simulink model "Accelero_Gyro_Combo_Lubins_Kalman"  (Simulink 7.0)
settings: Solver=FixedStepDiscrete  StartTime=0.0  StopTime=10.0  FixedStep=0.001  RelTol=1e-3
undefined symbols (not defined in the file or in its folder): Az, DiscIntNeverNeededParam, Kz, Ts
libraries: dsPICdrivers x6
settings Model: Creator=Lubin  LastModifiedBy=Prezes
settings OptimizationCC: OptimizeModelRefInitCode=on  LifeSpan=1
settings DebuggingCC: SaveWithParameterizedLinksMsg=none  SignalResolutionControl=TryResolveAllWithWarning
settings HardwareCC: ProdBitPerInt=16  ProdEndianess=LittleEndian  ProdWordSize=16  ProdHWDeviceType=16-bit Generic  TargetHWDeviceType=32-bit Generic
settings RTWCC: SystemTargetFile=dspic.tlc  TemplateMakefile=dspic_pic30_gcc.tmf  PostCodeGenCommand=dsPIC_Compile()  Description=Embedded Target for Microchip dsPIC (real-time)  ProcessScript=dspic_make_rtw_hook
settings CodeAppCC: IgnoreCustomStorageClasses=off
settings STFCustomTargetCC: GenFloatMathFcnCalls=ANSI_C  ModelReferenceCompliant=off  IncludeMdlTerminateFcn=off  CombineOutputUpdateFcns=on  SuppressErrorStatus=on  ERTCustomFileBanners=on  SupportContinuousTime=off  SupportNonInlinedSFcns=off  SystemTargetFile=dspic.tlc
settings ERTTargetCC: GenFloatMathFcnCalls=ANSI_C  ModelReferenceCompliant=off  CompOptLevelCompliant=off  IncludeMdlTerminateFcn=off  SuppressErrorStatus=on  ModelStepFunctionPrototypeControlCompliant=off  InlinedParameterPlacement=NonHierarchical  ERTSrcFileBannerTemplate=dsPIC_code_template.cgt  ERTHdrFileBannerTemplate=dsPIC_code_template.cgt  ERTDataSrcFileTemplate=dsPIC_code_template.cgt  ERTDataHdrFileTemplate=dsPIC_code_template.cgt  ERTCustomFileTemplate=dsPIC_main.tlc
settings CustomProperty: DataType=string  Value=D:\PROGRA~1\MATLAB\R2007b\bin\win32\gmake

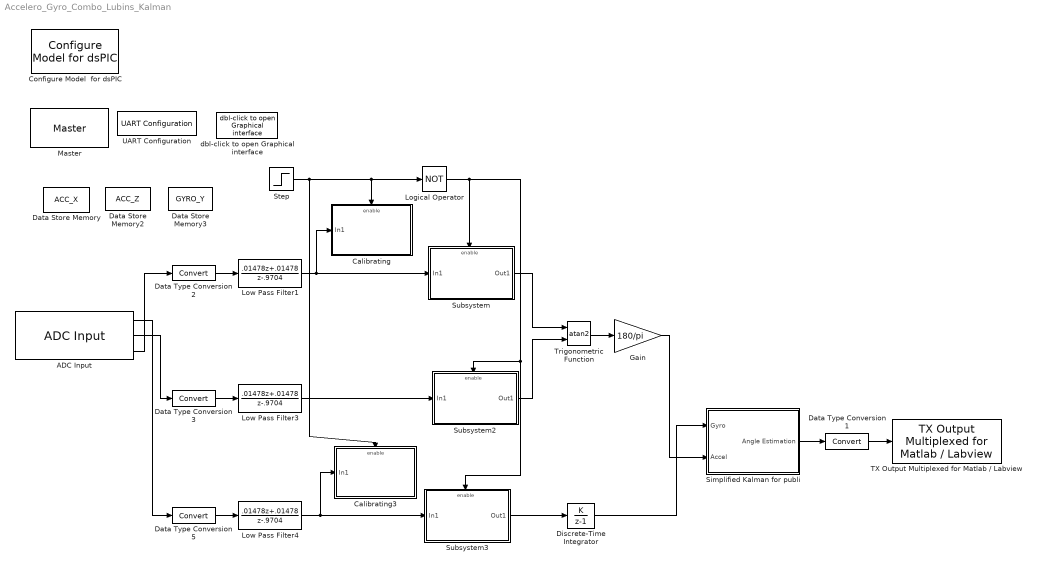
== system Accelero_Gyro_Combo_Lubins_Kalman ==
  ADC Input : dsPICdrivers/Peripheral I//O/ADC Input  Tag=dsPIC_ADC  Priority=5  ADC_TYPE=10 bits  ADC_MODE=Continuous sampling & get last channel value  NbrSampleStep=1  VoltRefpopup="AVdd  -  AVss"  OutFormatBitspopup=0000 00dd dddd dddd : Integer  InterruptPriority=6  ANCHANNELS=[11 14 15]  MaxName=ANmax = 1024  Rin=0  ADCS=3  SAMC=1  Temperature=25  DMAChannel=0  SampleTime=0.001  Status="OK  |  Tsmp=2.000e-007 |  T/Channel=2.600e-006 |  Tall=7.800e-006"
  Calibrating : Subsystem
  Calibrating3 : Subsystem
  Configure Model  for dsPIC : dsPICdrivers/Simulink Configuration/Configure Model  for dsPIC
  Data Store Memory : DataStoreMemory  DataStoreName=ACC_X  ReadBeforeWriteMsg=warning  WriteAfterWriteMsg=warning  WriteAfterReadMsg=warning  InitialValue=-1  OutDataType=sfix(16)  OutScaling=2^0
  Data Store Memory2 : DataStoreMemory  DataStoreName=ACC_Z  ReadBeforeWriteMsg=warning  WriteAfterWriteMsg=warning  WriteAfterReadMsg=warning  InitialValue=347  OutDataType=sfix(16)  OutScaling=2^0
  Data Store Memory3 : DataStoreMemory  DataStoreName=GYRO_Y  ReadBeforeWriteMsg=warning  WriteAfterWriteMsg=warning  WriteAfterReadMsg=warning  InitialValue=347  OutDataType=sfix(16)  OutScaling=2^0
  Data Type Conversion1 : DataTypeConversion  OutDataTypeMode=int16  OutDataType=sfix(16)  OutScaling=2^0
  Data Type Conversion2 : DataTypeConversion  OutDataTypeMode=double  OutDataType=sfix(16)  OutScaling=2^0
  Data Type Conversion3 : DataTypeConversion  OutDataTypeMode=double  OutDataType=sfix(16)  OutScaling=2^0
  Data Type Conversion5 : DataTypeConversion  OutDataTypeMode=double  OutDataType=sfix(16)  OutScaling=2^0
  Discrete-Time Integrator : DiscreteIntegrator  IntegratorMethod=Accumulation: Forward Euler  SampleTime=-1  OutDataTypeMode=double  OutDataType=sfix(16)  OutScaling=2^0  ICPrevOutput=DiscIntNeverNeededParam  ICPrevScaledInput=DiscIntNeverNeededParam
  Gain : Gain  Gain=180/pi  ParameterDataType=sfix(16)  ParameterScaling=2^0  OutDataTypeMode=double  OutDataType=sfix(16)  OutScaling=2^0
  Logical Operator : Logic  Operator=NOT  Inputs=1  AllPortsSameDT=off  OutDataTypeMode=boolean
  Low Pass Filter1 : DiscreteTransferFcn  Numerator=[.01478 .01478]  Denominator=[1 -.9704]  SampleTime=.001
  Low Pass Filter3 : DiscreteTransferFcn  Numerator=[.01478 .01478]  Denominator=[1 -.9704]  SampleTime=.001
  Low Pass Filter4 : DiscreteTransferFcn  Numerator=[.01478 .01478]  Denominator=[1 -.9704]  SampleTime=.001
  Master : dsPICdrivers/Master  Tag=dsPIC_MASTER  Priority=1  TimeStepType=Timer1  picType=30f6010A  fcy=10e6  Quartz_33f=5e6  PLLActive_33f=off  fcyDesired_33f=0  tmr1="[1  9999  0]"  tmr1Info="Time Step : 0.001  ;   Error : 0%  PR1=9999"  tmr2345="[0  0  0  0]"  tmr2345cfg=[-1 -1 -1 -1]  IOautoConf=on  typePort="[ 0  0  0  0  0  0  0  0  0  0  0  0  0  0  0  0  0  0  0  0  0  0  0  0  0  0  0  8  0  0  8  8  0  0  0  0  0  0  0  0  0  0  0  0  0  0  0  0  0  0  0  0  0  0  0  0  0  0  0  0  0  0  0  0  0  0  0  0  0  0  0  0  0  0  0  0  0  0  0  0  0  0  4  5  0  0  0  0  0  0  0  0  0  0  0  0  0  0  0  0  0  0  0  0  0  0  0  0  0  0  0  0 ]"  TRIS="[ 65535  65535  65535  65535  65535  65535  65535 ]"  ADPCFG=0  MasterBusyPort=None  MasterOverloadPort=None  FOSC=ECIO  TempProtection_33f=TEMP_ON  FPBOR=PBOR_OFF  PWRT=PWRT_OFF  MCLR=MCLR_DIS  PowerSave=off
  Simplified Kalman for publi : Subsystem
  Step : Step  Time=5  Before=1  After=0
  Subsystem : Subsystem
  Subsystem2 : Subsystem
  Subsystem3 : Subsystem
  TX Output Multiplexed for Matlab / Labview : dsPICdrivers/Serial PORT/TX Output Multiplexed for Matlab // Labview  Tag=dsPIC_TX_Multiplexed  Priority=5  UART=1  CleverSpreadingChk=on  CleverSpreading=1  CHANNEL=[0 ]  CHANNELBLOCKED=[]  CHANNELBLOCKED_BITEWISE=0  Status=OK
  Trigonometric Function : Trigonometry  Operator=atan2
  UART Configuration : dsPICdrivers/Serial PORT/UART Configuration  Tag=dsPIC_config_UART  Priority=2  UART=1  proposed_BAUD=9600  ALT_TX_RX=off  InterruptTxWhen=When Transmit Buffer is empty  TXInterruptPri=1  TxBufferSize=32  TXEN=on  InterruptRxWhen=When Receive Buffer is full (contain 4 characters)  RXInterruptPri=1  RxBufferSize=32  BAUD=9600  UxBRG=64  Info="UxBRG = 64   ||  Real Baud : 9615   ||  % error : 0.16026  ||  max 0.96154 Bytes / Step"  RealBaud=0
  dbl-click to open Graphical interface : dsPICdrivers/Serial PORT/dbl-click to open Graphical interface  SystemSampleTime=-1  Nothing=0
  wires:
  Trigonometric Function/1 -> Gain/1
  Discrete-Time Integrator/1 -> Simplified Kalman for publi/1(Gyro)
  Data Type Conversion2/1 -> Low Pass Filter1/1
  Low Pass Filter1/1 -> Calibrating/1(In1), Subsystem/1(In1)
  Step/1 -> Calibrating/Enable, Logical Operator/1, Calibrating3/Enable
  Logical Operator/1 -> Subsystem/Enable, Subsystem2/Enable, Subsystem3/Enable
  Data Type Conversion3/1 -> Low Pass Filter3/1
  Low Pass Filter3/1 -> Subsystem2/1(In1)
  Subsystem/1(Out1) -> Trigonometric Function/1
  Subsystem2/1(Out1) -> Trigonometric Function/2
  Data Type Conversion5/1 -> Low Pass Filter4/1
  Low Pass Filter4/1 -> Subsystem3/1(In1), Calibrating3/1(In1)
  Subsystem3/1(Out1) -> Discrete-Time Integrator/1
  ADC Input/3 -> Data Type Conversion2/1
  ADC Input/1 -> Data Type Conversion5/1
  ADC Input/2 -> Data Type Conversion3/1
  Gain/1 -> Simplified Kalman for publi/2(Accel)
  Simplified Kalman for publi/1(Angle Estimation) -> Data Type Conversion1/1
  Data Type Conversion1/1 -> TX Output Multiplexed for Matlab / Labview/1

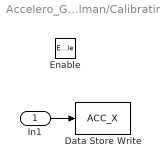
== system Accelero_Gyro_Combo_Lubins_Kalman/Calibrating ==
  In1 : Inport
  Enable : EnablePort  StatesWhenEnabling=reset
  Data Store Write : DataStoreWrite  DataStoreName=ACC_X  SampleTime=-1
  wires:
  In1/1 -> Data Store Write/1

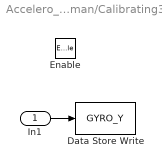
== system Accelero_Gyro_Combo_Lubins_Kalman/Calibrating3 ==
  In1 : Inport
  Enable : EnablePort  StatesWhenEnabling=reset
  Data Store Write : DataStoreWrite  DataStoreName=GYRO_Y  SampleTime=-1
  wires:
  In1/1 -> Data Store Write/1

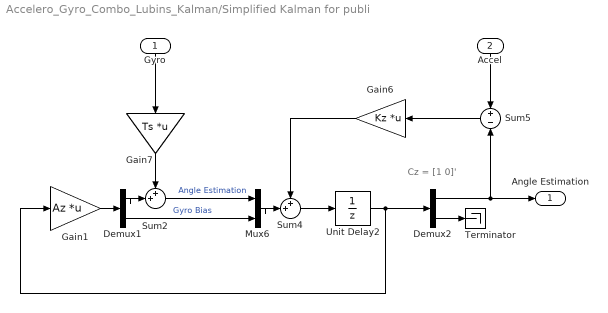
== system Accelero_Gyro_Combo_Lubins_Kalman/Simplified Kalman for publi ==
  note: Cz = [1 0]'
  Gyro : Inport  Orientation=down
  Accel : Inport  Orientation=down  Port=2
  Demux1 : Demux  Outputs=2
  Demux2 : Demux  Outputs=2
  Gain1 : Gain  Gain=Az  Multiplication=Matrix(K*u)  ParameterDataType=sfix(16)  ParameterScaling=2^0  OutDataType=sfix(16)  OutScaling=2^0
  Gain6 : Gain  Orientation=left  Gain=Kz  Multiplication=Matrix(K*u)  ParameterDataType=sfix(16)  ParameterScaling=2^0  OutDataType=sfix(16)  OutScaling=2^0
  Gain7 : Gain  Orientation=down  Gain=Ts  Multiplication=Matrix(K*u)  ParameterDataType=sfix(16)  ParameterScaling=2^0  OutDataType=sfix(16)  OutScaling=2^0
  Mux6 : Mux  Inputs=2
  Sum2 : Sum  Inputs=++|  OutDataType=sfix(16)  OutScaling=2^0
  Sum4 : Sum  Inputs=++|  OutDataType=sfix(16)  OutScaling=2^0
  Sum5 : Sum  Orientation=left  Inputs=+-  OutDataType=sfix(16)  OutScaling=2^0
  Terminator : Terminator
  Unit Delay2 : UnitDelay  SampleTime=-1
  Angle Estimation : Outport  OutDataType=sfix(16)  OutScaling=2^0
  wires:
  Gain6/1 -> Sum4/1
  Unit Delay2/1 -> Gain1/1, Demux2/1
  Gyro/1 -> Gain7/1
  Accel/1 -> Sum5/1
  Gain7/1 -> Sum2/1
  Sum5/1 -> Gain6/1
  Mux6/1 -> Sum4/2
  Demux1/2 -> Mux6/2  "Gyro Bias"
  Sum2/1 -> Mux6/1  "Angle Estimation"
  Demux1/1 -> Sum2/2
  Gain1/1 -> Demux1/1
  Demux2/1 -> Angle Estimation/1, Sum5/2
  Sum4/1 -> Unit Delay2/1
  Demux2/2 -> Terminator/1

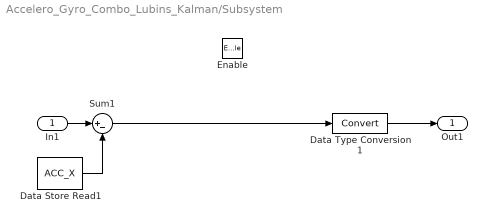
== system Accelero_Gyro_Combo_Lubins_Kalman/Subsystem ==
  In1 : Inport
  Enable : EnablePort  StatesWhenEnabling=reset
  Data Store Read1 : DataStoreRead  DataStoreName=ACC_X  SampleTime=-1
  Data Type Conversion1 : DataTypeConversion  OutDataTypeMode=double  OutDataType=sfix(16)  OutScaling=2^0
  Sum1 : Sum  Inputs=|+-  OutDataType=sfix(16)  OutScaling=2^0
  Out1 : Outport
  wires:
  Data Store Read1/1 -> Sum1/2
  Sum1/1 -> Data Type Conversion1/1
  Data Type Conversion1/1 -> Out1/1
  In1/1 -> Sum1/1

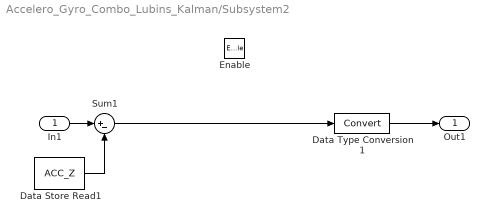
== system Accelero_Gyro_Combo_Lubins_Kalman/Subsystem2 ==
  In1 : Inport
  Enable : EnablePort  StatesWhenEnabling=reset
  Data Store Read1 : DataStoreRead  DataStoreName=ACC_Z  SampleTime=-1
  Data Type Conversion1 : DataTypeConversion  OutDataTypeMode=double  OutDataType=sfix(16)  OutScaling=2^0
  Sum1 : Sum  Inputs=|+-  OutDataType=sfix(16)  OutScaling=2^0
  Out1 : Outport
  wires:
  Data Store Read1/1 -> Sum1/2
  Sum1/1 -> Data Type Conversion1/1
  Data Type Conversion1/1 -> Out1/1
  In1/1 -> Sum1/1

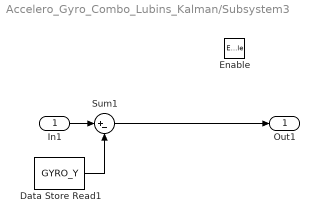
== system Accelero_Gyro_Combo_Lubins_Kalman/Subsystem3 ==
  In1 : Inport
  Enable : EnablePort  StatesWhenEnabling=reset
  Data Store Read1 : DataStoreRead  DataStoreName=GYRO_Y  SampleTime=-1
  Sum1 : Sum  Inputs=|+-  OutDataType=sfix(16)  OutScaling=2^0
  Out1 : Outport
  wires:
  In1/1 -> Sum1/1
  Sum1/1 -> Out1/1
  Data Store Read1/1 -> Sum1/2
